simulink library "battery_lib"  (R2018b)
settings: Solver=VariableStepAuto  StartTime=0.0  StopTime=10.0  RelTol=1e-3
values from neighbouring files (symbols this model uses):
  bat = batteryCreate('battery_params_default', 4, 4, C_rating, 3 )    [battery_example.m]
libraries: filters_lib x2
settings Model: Creator=Ybeyer  LastModifiedBy=yannic
settings DebuggingCC: LibraryContextMissingDiagnostic=none
settings SFSimCC: SimUseLocalCustomCode=off
settings RTWCC: RTWUseLocalCustomCode=off
settings CodeAppCC: StateflowObjectComments=on

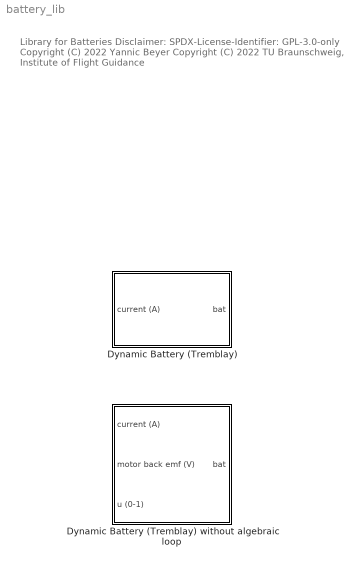
== system battery_lib ==
  note: Library for Batteries
      |
      | Disclaimer:
      | SPDX-License-Identifier: GPL-3.0-only
      |
      | Copyright (C) 2022 Yannic Beyer
      | Copyright (C) 2022 TU Braunschweig, Institute of Flight Guidance
  Dynamic Battery (Tremblay) : Subsystem  mask{bat=bat}
      mask prompts: bat "Battery parameters struct, see batteryCreate"
      mask Help: web('https://github.com/iff-gsc/LADAC/blob/main/propulsion/battery/README.md','-browser')
      mask DialogControl DescGroupVar Prompt: Dynamic Battery (Tremblay Model)
      mask DialogControl DescTextVar Prompt: Documentation here:
      mask DialogControl Control2 Prompt: README
      mask DialogControl Control2 Callback: web('https://github.com/iff-gsc/LADAC/blob/main/propulsion/battery/README.md','-browser')
  Dynamic Battery (Tremblay) without algebraic loop : Subsystem  mask{bat=bat, R_mot=0.001}
      mask prompts: bat "Battery parameters struct, see batteryCreate"; R_mot "Motor internal resistance, Ohm"
      mask Help: web('https://github.com/iff-gsc/LADAC/blob/main/propulsion/battery/README.md','-browser')
      mask DialogControl DescGroupVar Prompt: Dynamic Battery (Tremblay Model)
      mask DialogControl DescTextVar Prompt: Documentation here:
      mask DialogControl Control2 Prompt: README
      mask DialogControl Control2 Callback: web('https://github.com/iff-gsc/LADAC/blob/main/propulsion/battery/README.md','-browser')

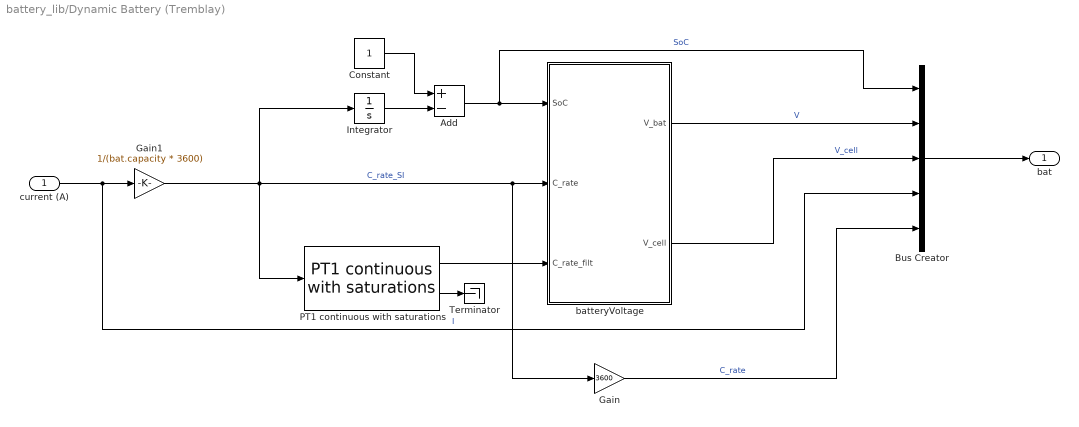
== system battery_lib/Dynamic Battery (Tremblay) ==
  current (A) : Inport
  Add : Sum  Inputs=+-
  Bus Creator : BusCreator  Inputs=5
  Constant : Constant
  Gain : Gain  Gain=3600
  Gain1 : Gain  Gain=1/(bat.capacity * 3600)
  Integrator : Integrator
  PT1 continuous with saturations : filters_lib/PT1 continuous with saturations  T=bat.tc  x_max=inf  x_min=-inf  x_dt_max=inf  x_dt_min=-inf  x_init=0
      settings: SourceProductName=LADAC
  Terminator : Terminator
  batteryVoltage : MATLAB Function  TreatAsAtomicUnit=on
  bat : Outport
  wires:
  batteryVoltage/1(V_bat) -> Bus Creator/2  "V"
  PT1 continuous with saturations/1 -> batteryVoltage/3(C_rate_filt)
  PT1 continuous with saturations/2 -> Terminator/1
  Integrator/1 -> Add/2
  Add/1 -> Bus Creator/1, batteryVoltage/1(SoC)  "SoC"
  Constant/1 -> Add/1
  Bus Creator/1 -> bat/1
  current (A)/1 -> Bus Creator/4, Gain1/1  "I"
  Gain1/1 -> PT1 continuous with saturations/1, Integrator/1, Gain/1, batteryVoltage/2(C_rate)  "C_rate_SI"
  Gain/1 -> Bus Creator/5  "C_rate"
  batteryVoltage/2(V_cell) -> Bus Creator/3  "V_cell"

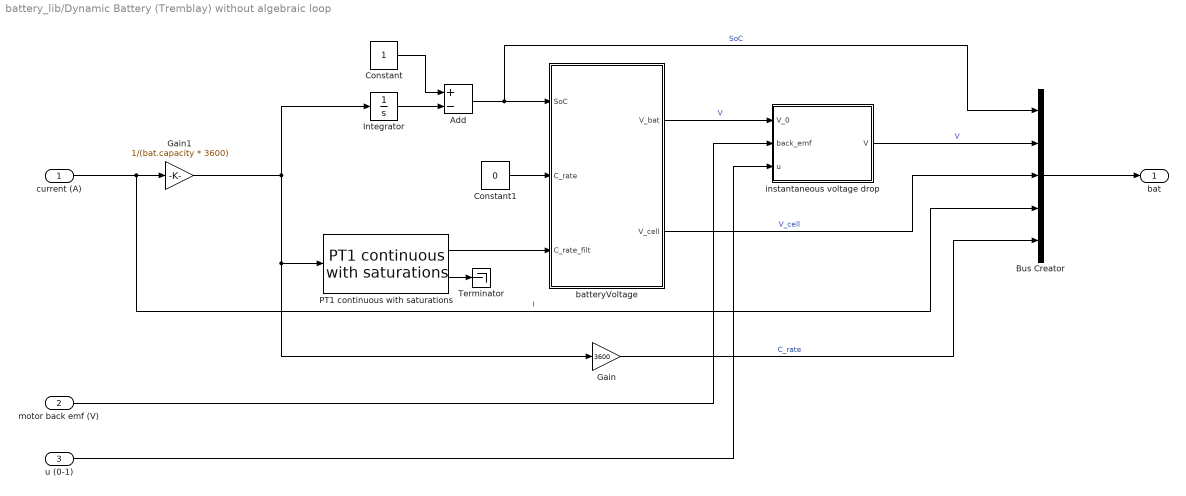
== system battery_lib/Dynamic Battery (Tremblay) without algebraic loop ==
  current (A) : Inport
  motor back emf (V) : Inport  Port=2
  u (0-1) : Inport  Port=3
  Add : Sum  Inputs=+-
  Bus Creator : BusCreator  Inputs=5
  Constant : Constant
  Constant1 : Constant  Value=0
  Gain : Gain  Gain=3600
  Gain1 : Gain  Gain=1/(bat.capacity * 3600)
  Integrator : Integrator
  PT1 continuous with saturations : filters_lib/PT1 continuous with saturations  T=bat.tc  x_max=inf  x_min=-inf  x_dt_max=inf  x_dt_min=-inf  x_init=0
      settings: SourceProductName=LADAC
  Terminator : Terminator
  batteryVoltage : MATLAB Function  TreatAsAtomicUnit=on
  instantaneous voltage drop : MATLAB Function  TreatAsAtomicUnit=on
  bat : Outport
  wires:
  batteryVoltage/2(V_cell) -> Bus Creator/3  "V_cell"
  Gain/1 -> Bus Creator/5  "C_rate"
  Gain1/1 -> Gain/1, PT1 continuous with saturations/1, Integrator/1
  current (A)/1 -> Gain1/1, Bus Creator/4  "I"
  Bus Creator/1 -> bat/1
  Constant/1 -> Add/1
  Add/1 -> batteryVoltage/1(SoC), Bus Creator/1  "SoC"
  Integrator/1 -> Add/2
  PT1 continuous with saturations/2 -> Terminator/1
  PT1 continuous with saturations/1 -> batteryVoltage/3(C_rate_filt)
  batteryVoltage/1(V_bat) -> instantaneous voltage drop/1(V_0)  "V"
  Constant1/1 -> batteryVoltage/2(C_rate)
  instantaneous voltage drop/1(V) -> Bus Creator/2  "V"
  motor back emf (V)/1 -> instantaneous voltage drop/2(back_emf)
  u (0-1)/1 -> instantaneous voltage drop/3(u)

== matlab function battery_lib/Dynamic Battery (Tremblay) without algebraic loop/instantaneous voltage drop ==
  data: V_0 input; back_emf input; u input; V output; bat parameter; R_mot parameter
function V = fcn(V_0,back_emf,u,bat, R_mot)
R_bat = bat.R_times_C / (bat.capacity * 3600) * bat.num_serial;
V = (V_0+R_bat*sum(back_emf./R_mot))./(1+R_bat*sum(u./R_mot));
end

== matlab function battery_lib/Dynamic Battery (Tremblay)/batteryVoltage ==
  data: bat parameter; SoC input; V_bat output; C_rate input; C_rate_filt input; V_cell output
function [V_bat,V_cell] = batteryVoltage(bat,SoC,C_rate,C_rate_filt)
[V_bat,V_cell] = batteryVoltage(bat,SoC,C_rate,C_rate_filt);
end

== matlab function battery_lib/Dynamic Battery (Tremblay) without algebraic loop/batteryVoltage ==
  data: bat parameter; SoC input; V_bat output; C_rate input; C_rate_filt input; V_cell output
function [V_bat,V_cell] = batteryVoltage(bat,SoC,C_rate,C_rate_filt)
[V_bat,V_cell] = batteryVoltage(bat,SoC,C_rate,C_rate_filt);
end
